simulink model "ControlLogic_Testrig"  (R2025a)
settings: Solver=ode3  StartTime=0.0  StopTime=20  FixedStep=0.001  MaxStep=1e-4  RelTol=1e-3  EnableMultiTasking=on
undefined symbols (not defined in the file): sigbuilder_block
Description:
  | Copyright 2014-2025 MathWorks, Inc.
settings Model: MinMaxOverflowLogging=ForceOff  Creator=smiller  LastModifiedBy=smiller
settings SolverCC: AlgebraicLoopSolver=TrustRegion
settings DataIOCC: LimitDataPoints=on  SaveFormat=Array  SignalLoggingSaveFormat=ModelDataLogs  ReturnWorkspaceOutputs=off
settings OptimizationCC: ReuseModelBlockBuffer=off  ExpressionDepthLimit=2147483647.0  LifeSpan=inf
settings DebuggingCC: UnderspecifiedInitializationDetection=Classic  MergeDetectMultiDrivingBlocksExec=none  FcnCallInpInsideContextMsg=warning  UnconnectedInputMsg=warning  UnconnectedOutputMsg=warning  UnconnectedLineMsg=warning  AllowSymbolicDim=off  StateNameClashWarn=warning  PregeneratedLibrarySubsystemCodeDiagnostic=none  SFUnexpectedBacktrackingDiag=warning  SFNoUnconditionalDefaultTransitionDiag=warning  SFExecutionAtInitializationDiag=none  ArithmeticOperatorsInVariantConditions=warning
settings HardwareCC: ProdBitPerPointer=32.0  ProdBitPerSizeT=32.0  ProdBitPerPtrDiffT=32.0  ProdLargestAtomicFloat=None  ProdIntDivRoundTo=Undefined  ProdEndianess=Unspecified  ProdWordSize=32.0  ProdHWDeviceType=32-bit Generic
settings ModelReferenceCC: EnableRefExpFcnMdlSchedulingChecks=on  PropagateSignalLabelsOutOfModel=off
settings SFSimCC: SimUseLocalCustomCode=off  SimParseCustomCode=off  CustomCodeUndefinedFunction=UseInterfaceOnly
settings RTWCC: RTWUseLocalCustomCode=off  GPUComputeCapability=3.5  DLArmComputeVersion=19.05
settings CodeAppCC: StateflowObjectComments=on
settings GRTTargetCC: TargetLangStandard=C89/C90 (ANSI)  CombineOutputUpdateFcns=off  GRTInterface=on
settings ConfigComp: CovEnable=on  CovScope=ReferencedModels  CovIncludeTopModel=off  CovMetricSettings=dcm  CovHTMLOptions=-sRT=1 -sVT=0 -aTS=1 -bRG=1 -bTC=1 -hTR=0 -nFC=0 -nFD=1 -scm=1 -bcm=1 -xEv=0 -xEM=0  CovSaveCumulativeToWorkspaceVar=on  CovCumulativeVarName=cvdata_ControlLogic_Testrig  CovModelRefEnable=all  CovExternalEMLEnable=off  CovSFcnEnable=off  DVMaxProcessTime=300.0  DVModelCoverageObjectives=MCDC  DVMaxTestCaseSteps=500.0  DVTestSuiteOptimization=Auto  DVIgnoreCovSatisfied=on  DVCoverageDataFile=cvdata_ControlLogic_Testrig.cvt  DVAbsoluteTolerance=1.0e-5  DVDefectChecker=off  DVMaxViolationSteps=20.0  DVHarnessSource=Signal Editor  DVRebuildModelRepresentation=Always  DVActiveTab=0.0

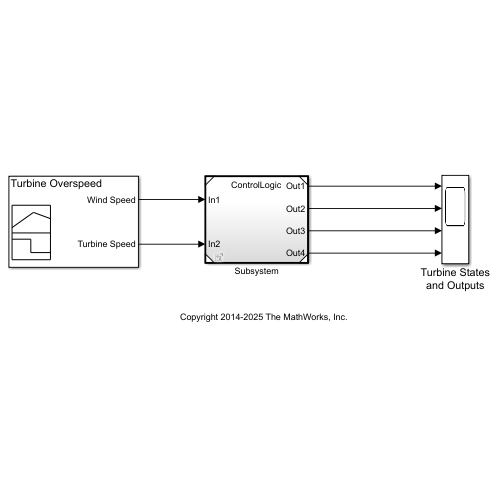
[thumbnail: Simulink's stored preview of the top-level diagram]
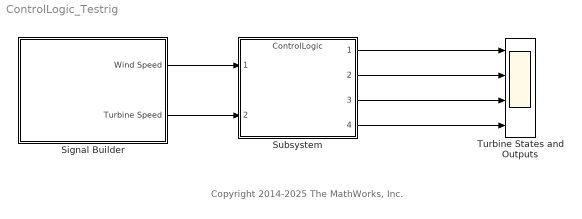
== system ControlLogic_Testrig ==
  note: Copyright 2014-2025 The MathWorks, Inc.
  Signal Builder : Subsystem  Tag=STV Subsys  LoadFcn=sigbuilder_block('load',[316.5 171.75 805.5 485.25 ]);  StartFcn=sigbuilder_block('start');  StopFcn=sigbuilder_block('stop');  ClipboardFcn=sigbuilder_block('clipboard');  mask(Sigbuilder block){tuvar=[0:10]}
      mask help: Sigbuilder GUI
      mask init:
      | if ~strcmp(get_param(bdroot(gcbh),'SimulationStatus'),'stopped') tuvar = sigbuilder_block('maskInit'); end
      settings: CopyFcn=sigbuilder_block('copy');  DeleteFcn=sigbuilder_block('delete');  ModelCloseFcn=sigbuilder_block('modelClose');  PreSaveFcn=sigbuilder_block('preSave');  PauseFcn=sigbuilder_block('pause')  ContinueFcn=sigbuilder_block('continue')  NameChangeFcn=sigbuilder_block('namechange');  OpenFcn=sigbuilder_block('open',[3 32.25 762 490.5 ]);  CloseFcn=sigbuilder_block('close');
      mask Display: plot(0, 0, 100, 100,[2, 2, 32, 32, 2], [68, 8, 8, 68, 68],[32, 2], [38, 38], [32, 19, 2],[53, 60, 44], [32, 17, 17, 2],[16, 16, 31, 31]);txt = getActiveGroup(gcbh);text(2, 100, txt,'verticalAlignment', 'top');
  Subsystem : ModelReference  ModelNameDialog=ControlLogic.slx  SimulationMode=Normal  ModelReferenceVersion=10.1
  Turbine States and Outputs : Scope  NumInputPorts=4
      settings: ActiveDisplayYMinimum=-5  ActiveDisplayYMaximum=5
  wires:
  Signal Builder/1(Wind Speed) -> Subsystem/1
  Signal Builder/2(Turbine Speed) -> Subsystem/2
  Subsystem/1 -> Turbine States and Outputs/1
  Subsystem/2 -> Turbine States and Outputs/2
  Subsystem/3 -> Turbine States and Outputs/3
  Subsystem/4 -> Turbine States and Outputs/4

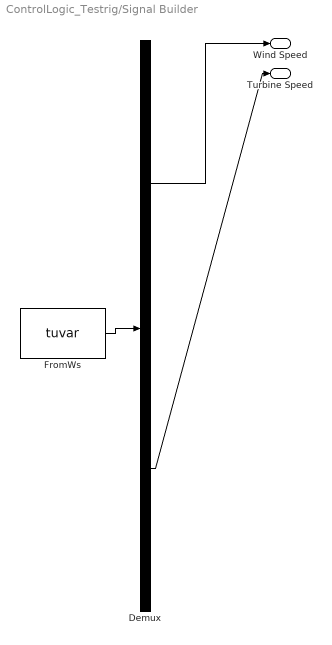
== system ControlLogic_Testrig/Signal Builder ==
  Demux : Demux  Tag=STV Demux  Outputs=2
      settings: DisplayOption=none
  FromWs : FromWorkspace  Tag=STV FromWs  VariableName=tuvar
      SigBuilderData=|
      | common.afterFinalStr = 'Extrapolate'
      | common.sampleTime = 0
      | dataSet(1).timeRange = [0 20]
      | dataSet(1).name = 'Simple Start and Stop'
      | dataSet(2).timeRange = [0 20]
      | dataSet(2).name = 'High Winds'
      | dataSet(3).timeRange = [0 20]
      | dataSet(3).name = 'Turbine Overspeed'
      | sbobj.Groups(1).Name = 'Simple Start and Stop'
      | sbobj.Groups(1).Signals(1).Name = 'Wind Speed'
      | sbobj.Groups(1).Signals(1).XData = [0 6 8.66 14 20]
      | sbobj.Groups(1).Signals(1).YData = [0 10 10 0 0]
      | sbobj.Groups(1).Signals(2).Name = 'Turbine Speed'
      | sbobj.Groups(1).Signals(2).XData = [0 4.42 4.42 6.46 10.02 16 20]
      | sbobj.Groups(1).Signals(2).YData = [0 0 0.37 1800 1800 0 0]
      | sbobj.Groups(1).TimeRange = [0 20]
      | sbobj.Groups(2).Name = 'High Winds'
      | sbobj.Groups(2).Signals(1).Name = 'Wind Speed'
      | sbobj.Groups(2).Signals(1).XData = [0 4 6 8.66 20]
      | sbobj.Groups(2).Signals(1).YData = [0 10 10 22 22]
      | sbobj.Groups(2).Signals(2).Name = 'Turbine Speed'
      | sbobj.Groups(2).Signals(2).XData = [0 4.42 4.42 6.46 10.02 11.98 11.98 20]
      | sbobj.Groups(2).Signals(2).YData = [0 0 0.37 1800 1800 20 0 0]
      | sbobj.Groups(2).TimeRange = [0 20]
      | sbobj.Groups(3).Name = 'Turbine Overspeed'
      | sbobj.Groups(3).Signals(1).Name = 'Wind Speed'
      | sbobj.Groups(3).Signals(1).XData = [0 4 6 8.66 14.85 20]
      | sbobj.Groups(3).Signals(1).YData = [0 10 10 12 12 12]
      | sbobj.Groups(3).Signals(2).Name = 'Turbine Speed'
      | sbobj.Groups(3).Signals(2).XData = [0 4.42 4.42 6.46 10.02 11.98 15.5 18.94 20]
      | sbobj.Groups(3).Signals(2).YData = [0 0 0.37 1800 1800 2200 2200 0 0]
      | sbobj.Groups(3).TimeRange = [0 20]
  Wind Speed : Outport  Tag=STV Outport  VectorParamsAs1DForOutWhenUnconnected=off
  Turbine Speed : Outport  Tag=STV Outport  Port=2  VectorParamsAs1DForOutWhenUnconnected=off
  wires:
  Demux/1 -> Wind Speed/1
  FromWs/1 -> Demux/1
  Demux/2 -> Turbine Speed/1
